simulink model "Bsw_PMSMCtrl_SimInput"  (R2023b)
settings: Solver=FixedStepDiscrete  StartTime=0.0  StopTime=0.3  RelTol=1e-3
PreLoadFcn:
  | addpath("Sim\")
  | Sim_PreLoad_PMSMCtrl;
values from neighbouring files (symbols this model uses):
  Par_Mtr_cuNp = 5    [Sw_PMSMCtrl.sldd]
libraries: simulink x1
settings Model: Creator=62555  LastModifiedBy=62555
settings OptimizationCC: DefaultParameterBehavior=Inlined  UseDivisionForNetSlopeComputation=on  DefaultUnderspecifiedDataType=single  EnhancedBackFolding=on  PassReuseOutputArgsAs=Individual arguments  ZeroExternalMemoryAtStartup=off  ZeroInternalMemoryAtStartup=off  OptimizeBlockOrder=speed  DifferentSizesBufferReuse=on  OptimizationCustomize=off  EfficientTunableParamExpr=on
settings DebuggingCC: ParameterPrecisionLossMsg=none  ParameterTunabilityLossMsg=error
settings SFSimCC: MATLABDynamicMemAlloc=off
settings RTWCC: Description=Embedded Coder  SystemTargetFile=ert.tlc  GenCodeOnly=on  TemplateMakefile=ert_default_tmf  GenerateReport=on  LaunchReport=on
settings CodeAppCC: ForceParamTrailComments=on  IgnoreCustomStorageClasses=off  OperatorAnnotations=on  SimulinkDataObjDesc=on  SFDataObjDesc=on  InsertBlockDesc=on
settings ERTTargetCC: TargetLangStandard=C99 (ISO)  GenerateSampleERTMain=on  InlinedParameterPlacement=NonHierarchical  ERTCustomFileTemplate=example_file_process.tlc

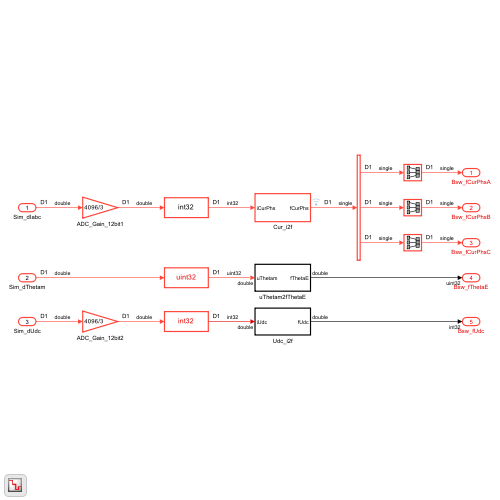
[thumbnail: Simulink's stored preview of the top-level diagram]
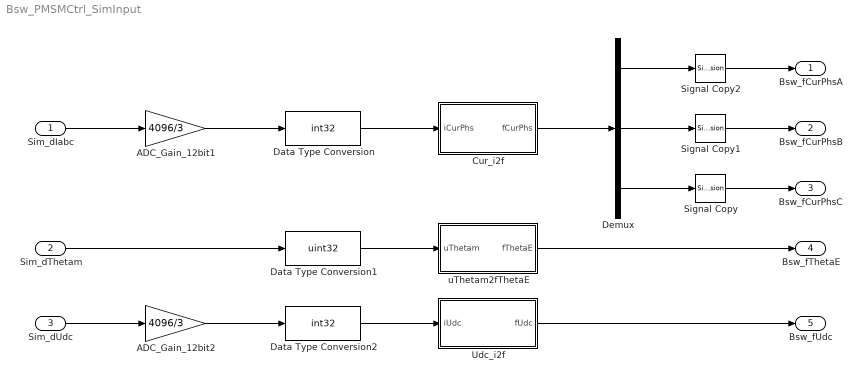
== system Bsw_PMSMCtrl_SimInput ==
  Sim_dIabc : Inport  OutDataTypeStr=double
  Sim_dThetam : Inport  Port=2  OutDataTypeStr=double
  Sim_dUdc : Inport  Port=3  OutDataTypeStr=double
  ADC_Gain_12bit1 : Gain  Gain=4096/3
  ADC_Gain_12bit2 : Gain  Gain=4096/3
  Cur_i2f : Subsystem  RTWFileName=Lib_Local
      settings: RTWFcnNameOpts=Use subsystem name  RTWFileNameOpts=User specified
  Data Type Conversion : DataTypeConversion  OutDataTypeStr=int32  SaturateOnIntegerOverflow=off  RndMeth=Floor
  Data Type Conversion1 : DataTypeConversion  OutDataTypeStr=uint32  SaturateOnIntegerOverflow=off  RndMeth=Floor
  Data Type Conversion2 : DataTypeConversion  OutDataTypeStr=int32  SaturateOnIntegerOverflow=off  RndMeth=Floor
  Demux : Demux  Outputs=3
  Signal Copy : SignalConversion  OverrideOpt=off
  Signal Copy1 : SignalConversion  OverrideOpt=off
  Signal Copy2 : SignalConversion  OverrideOpt=off
  Udc_i2f : Subsystem  TreatAsAtomicUnit=on
      settings: RTWSystemCode=Nonreusable function  RTWFcnNameOpts=Use subsystem name  FunctionInterfaceSpec=Allow arguments (Optimized)
  uThetam2fThetaE : Subsystem  TreatAsAtomicUnit=on
      settings: RTWSystemCode=Nonreusable function  RTWFcnNameOpts=Use subsystem name  FunctionInterfaceSpec=Allow arguments (Optimized)
  Bsw_fCurPhsA : Outport
  Bsw_fCurPhsB : Outport  Port=2
  Bsw_fCurPhsC : Outport  Port=3
  Bsw_fThetaE : Outport  Port=4
  Bsw_fUdc : Outport  Port=5
  wires:
  Data Type Conversion2/1 -> Udc_i2f/1(iUdc)
  Sim_dUdc/1 -> ADC_Gain_12bit2/1
  Sim_dThetam/1 -> Data Type Conversion1/1
  Data Type Conversion/1 -> Cur_i2f/1(iCurPhs)
  Data Type Conversion1/1 -> uThetam2fThetaE/1(uThetam)
  Sim_dIabc/1 -> ADC_Gain_12bit1/1
  ADC_Gain_12bit1/1 -> Data Type Conversion/1
  ADC_Gain_12bit2/1 -> Data Type Conversion2/1
  Cur_i2f/1(fCurPhs) -> Demux/1
  Demux/1 -> Signal Copy2/1
  Demux/2 -> Signal Copy1/1
  Demux/3 -> Signal Copy/1
  Signal Copy/1 -> Bsw_fCurPhsC/1
  Signal Copy1/1 -> Bsw_fCurPhsB/1
  Signal Copy2/1 -> Bsw_fCurPhsA/1
  uThetam2fThetaE/1(fThetaE) -> Bsw_fThetaE/1
  Udc_i2f/1(fUdc) -> Bsw_fUdc/1

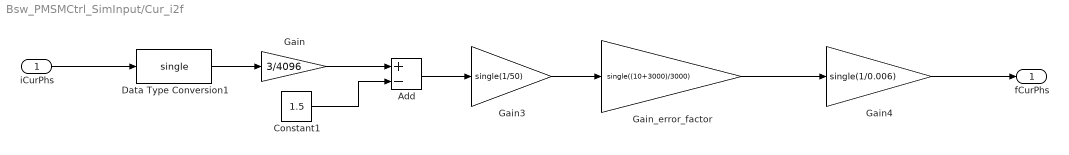
== system Bsw_PMSMCtrl_SimInput/Cur_i2f ==
  iCurPhs : Inport
  Add : Sum  Inputs=+-
  Constant1 : Constant  Value=1.5  OutDataTypeStr=single  SampleTime=-1
  Data Type Conversion1 : DataTypeConversion  OutDataTypeStr=single  SaturateOnIntegerOverflow=off  RndMeth=Floor
  Gain : Gain  Gain=3/4096
  Gain3 : Gain  Gain=single(1/50)  OutDataTypeStr=Inherit: Same as input
  Gain4 : Gain  Gain=single(1/0.006)
  Gain_error_factor : Gain  Gain=single((10+3000)/3000)
  fCurPhs : Outport
  wires:
  Gain_error_factor/1 -> Gain4/1
  Gain3/1 -> Gain_error_factor/1
  Data Type Conversion1/1 -> Gain/1
  iCurPhs/1 -> Data Type Conversion1/1
  Gain/1 -> Add/1
  Constant1/1 -> Add/2
  Gain4/1 -> fCurPhs/1
  Add/1 -> Gain3/1

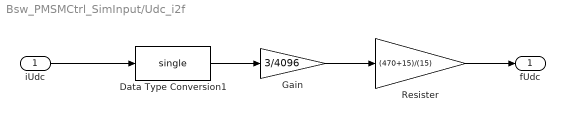
== system Bsw_PMSMCtrl_SimInput/Udc_i2f ==
  iUdc : Inport
  Data Type Conversion1 : DataTypeConversion  OutDataTypeStr=single  SaturateOnIntegerOverflow=off  RndMeth=Floor
  Gain : Gain  Gain=3/4096
  Resister : Gain  Gain=(470+15)/(15)
  fUdc : Outport
  wires:
  Resister/1 -> fUdc/1
  Gain/1 -> Resister/1
  iUdc/1 -> Data Type Conversion1/1
  Data Type Conversion1/1 -> Gain/1

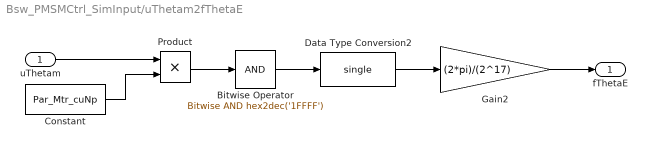
== system Bsw_PMSMCtrl_SimInput/uThetam2fThetaE ==
  uThetam : Inport
  Bitwise Operator : simulink/Logic and Bit Operations/Bitwise Operator  logicop=AND  UseBitMask=on  BitMask=hex2dec('1FFFF')  BitMaskRealWorld=Stored Integer
  Constant : Constant  Value=Par_Mtr_cuNp  OutDataTypeStr=uint32  SampleTime=-1
  Data Type Conversion2 : DataTypeConversion  OutDataTypeStr=single  SaturateOnIntegerOverflow=off  RndMeth=Floor
  Gain2 : Gain  Gain=(2*pi)/(2^17)
  Product : Product  OutDataTypeStr=uint32
  fThetaE : Outport
  wires:
  uThetam/1 -> Product/1
  Product/1 -> Bitwise Operator/1
  Bitwise Operator/1 -> Data Type Conversion2/1
  Data Type Conversion2/1 -> Gain2/1
  Gain2/1 -> fThetaE/1
  Constant/1 -> Product/2
